simulink model "ABS"  (R2023b)
settings: Solver=FixedStepAuto  StartTime=0.0  StopTime=10  FixedStep=1e-3  MaxStep=1e-3  RelTol=1e-3
values from neighbouring files (symbols this model uses):
  B = 10    [Parameters.m]
  C = 1.9    [Parameters.m]
  D = 1.0    (= 1)    [Parameters.m]
  E = 0.97    [Parameters.m]
  effR = 0.30    (= 0.3)    [Parameters.m]
  g = 9.81    [Parameters.m]
  Jw = 1.8    [Parameters.m]
  lambda_ref = 0.20    (= 0.2)    [Parameters.m]
  omega0 = v0 / effR    (= 92.6)    [Parameters.m]
  QuarterCarMass = 350    [Parameters.m]
  tau_b = 0.03    [Parameters.m]
  Tmax = 2000    [Parameters.m]
  v0 = 27.78    [Parameters.m]
  v_epsilon = 0.5    [Parameters.m]
libraries: slpidlib x1
settings Model: Creator=SEIF  LastModifiedBy=SEIF

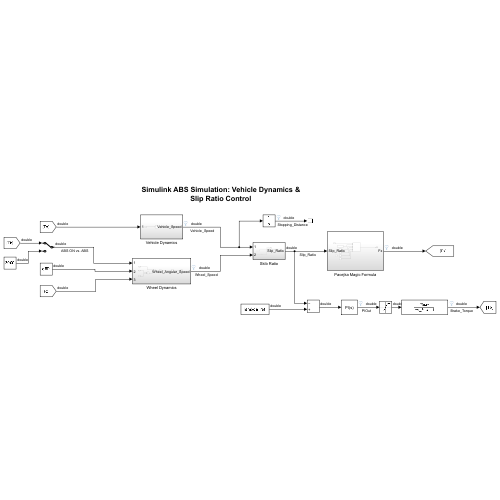
[thumbnail: Simulink's stored preview of the top-level diagram]
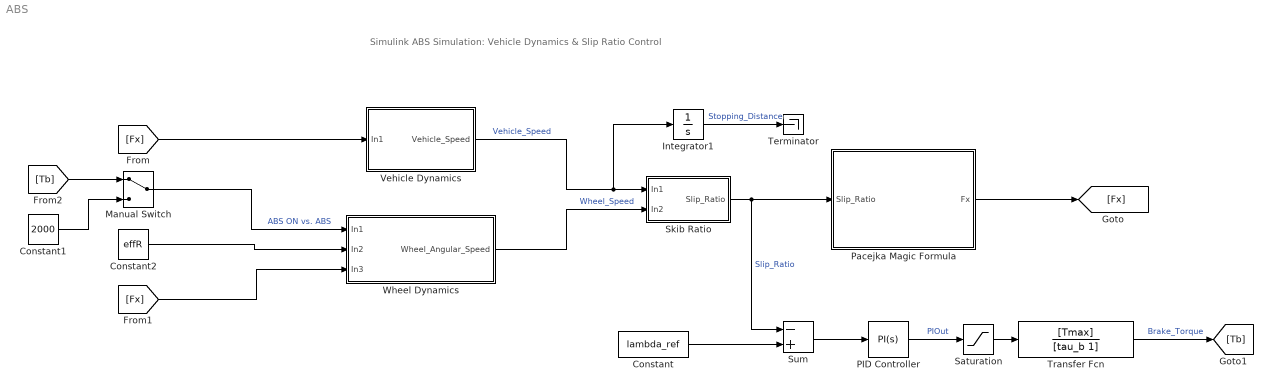
== system ABS ==
  note: Simulink ABS Simulation: Vehicle Dynamics & Slip Ratio Control
  Constant : Constant  Value=lambda_ref
  Constant1 : Constant  Value=2000
  Constant2 : Constant  Value=effR
  Integrator1 : Integrator
  Manual Switch : ManualSwitch
  PID Controller : slpidlib/PID Controller  Controller=PI  Form=Parallel  TimeDomain=Continuous-time  UseExternalTs=off  SampleTime=-1  IntegratorMethod=Forward Euler  FilterMethod=Forward Euler  ControllerParametersSource=internal  P=100  I=10  UseKiTs=off  D=0  N=100  UseFilter=on  TunerSelectOption=Transfer Function Based (PID Tuner App)  InitialConditionSource=internal  InitialConditionForIntegrator=0  InitialConditionForFilter=0  DifferentiatorICPrevScaledInput=0  ExternalReset=none  TrackingMode=off  Kt=1  LimitOutput=off  SatLimitsSource=internal  UpperSaturationLimit=inf  LowerSaturationLimit=-inf  LinearizeAsGain=on  AntiWindupMode=none  Kb=1  LimitIntegrator=off  UpperIntegratorSaturationLimit=inf  LowerIntegratorSaturationLimit=-inf  POutMin=[]  POutMax=[]  IOutMin=[]  IOutMax=[]  DOutMin=[]  DOutMax=[]  NOutMin=[]  NOutMax=[]  SumOutMin=[]  SumOutMax=[]  SaturationOutMin=[]  SaturationOutMax=[]  PParamMin=[]  PParamMax=[]  IParamMin=[]  IParamMax=[]  DParamMin=[]  DParamMax=[]  NParamMin=[]  NParamMax=[]  KbParamMin=[]  KbParamMax=[]  KtParamMin=[]  KtParamMax=[]  KbOutMin=[]  KbOutMax=[]  KtOutMin=[]  KtOutMax=[]  IntegratorOutMin=[]  IntegratorOutMax=[]  FilterOutMin=[]  FilterOutMax=[]  SumI1OutMin=[]  SumI1OutMax=[]  SumI2OutMin=[]  SumI2OutMax=[]  SumI3OutMin=[]  SumI3OutMax=[]  SumI4OutMin=[]  SumI4OutMax=[]  SumDOutMin=[]  SumDOutMax=[]  DifferentiatorOutMin=[]  DifferentiatorOutMax=[]  FilterDiffOutCoefMin=[]  FilterDiffOutCoefMax=[]  ReciprocalOutMin=[]  ReciprocalOutMax=[]  SumDenOutMin=[]  SumDenOutMax=[]  SumNumOutMin=[]  SumNumOutMax=[]  DivideOutMin=[]  DivideOutMax=[]  UdiffTsProdOutMin=[]  UdiffTsProdOutMax=[]  NTsProdOutMin=[]  NTsProdOutMax=[]  UintegralTsProdOutMin=[]  UintegralTsProdOutMax=[]  UngainTsProdOutMin=[]  UngainTsProdOutMax=[]  ClampingZeroOutDataTypeStr=Inherit: Inherit via back propagation  ClampingZeroOutMin=[]  ClampingZeroOutMax=[]  FilterDenConstantOutDataTypeStr=Inherit: Inherit via back propagation  FilterDenConstantOutMin=[]  FilterDenConstantOutMax=[]  PCopyOutDataTypeStr=Inherit: Inherit via back propagation  PCopyOutMin=[]  PCopyOutMax=[]  NCopyOutDataTypeStr=Inherit: Inherit via back propagation  NCopyOutMin=[]  NCopyOutMax=[]  IntegratorContinuousStateAttributes=''  IntegratorStateMustResolveToSignalObject=off  IntegratorRTWStateStorageClass=Auto  FilterContinuousStateAttributes=''  FilterStateMustResolveToSignalObject=off  FilterRTWStateStorageClass=Auto  ParallelPVariant=InternalParameters  IdealPVariant=Disabled  IVariant=InternalParameters  DVariant=Disabled  IntegratorVariant=Continuous  SatVariant=Disabled  AWVariant=Passthrough  PCopyVariant=Disabled  TRVariant=Disabled  FdbkBlocksVariant=Forward  IdealPFdbkVariant=Disabled  SatFdbkVariant=Disabled  DerivativeFilterVariant=Disabled  NVariant=Disabled  NCopyVariant=Disabled_SignalSpec  FilterICVariant=Disabled  IntegratorICVariant=InternalICs  ExternalResetVariant=Disabled  TRSumVariant=Passthrough  SumFdbkVariant=Disabled  SumVariant=Sum_PI  TsampFilterVariant=InternalTs  TsampNgainVariant=Passthrough  TsampIntegralVariant=Disabled_SignalSpec  ExternalSaturationOutDataTypeStr=Inherit: Same as second input
  Pacejka Magic Formula : Subsystem
  Saturation : Saturate  UpperLimit=1  LowerLimit=0
  Skib Ratio : Subsystem
  Sum : Sum  Inputs=-+
  Terminator : Terminator
  Transfer Fcn : TransferFcn  Numerator=[Tmax]  Denominator=[tau_b 1]
  Vehicle Dynamics : Subsystem
  Wheel Dynamics : Subsystem
  wires:
  Pacejka Magic Formula/1(Fx) -> [Fx]
  Constant2/1 -> Wheel Dynamics/2(In2)
  [Fx] -> Wheel Dynamics/3(In3)
  [Fx] -> Vehicle Dynamics/1(In1)
  Wheel Dynamics/1(Wheel_Angular_Speed) -> Skib Ratio/2(In2)  "Wheel_Speed"
  Skib Ratio/1(Slip_Ratio) -> Sum/1, Pacejka Magic Formula/1(Slip_Ratio)  "Slip_Ratio"
  Constant/1 -> Sum/2
  Sum/1 -> PID Controller/1
  PID Controller/1 -> Saturation/1  "PIOut"
  Saturation/1 -> Transfer Fcn/1
  Transfer Fcn/1 -> [Tb]  "Brake_Torque"
  Integrator1/1 -> Terminator/1  "Stopping_Distance"
  Vehicle Dynamics/1(Vehicle_Speed) -> Integrator1/1, Skib Ratio/1(In1)  "Vehicle_Speed"
  Manual Switch/1 -> Wheel Dynamics/1(In1)  "ABS ON vs. ABS"
  [Tb] -> Manual Switch/1
  Constant1/1 -> Manual Switch/2

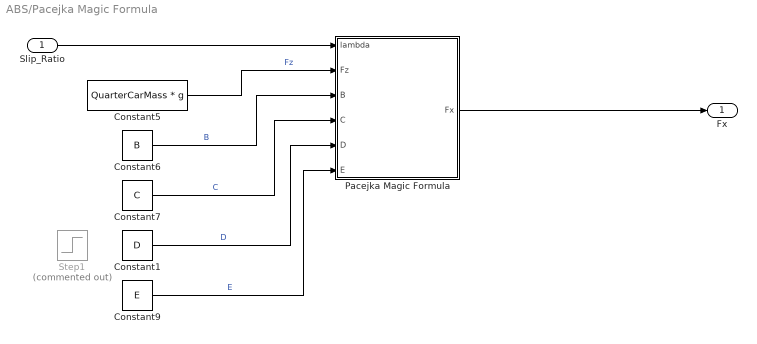
== system ABS/Pacejka Magic Formula ==
  Slip_Ratio : Inport
  Constant1 : Constant  Value=D
  Constant5 : Constant  Value=QuarterCarMass * g
  Constant6 : Constant  Value=B
  Constant7 : Constant  Value=C
  Constant9 : Constant  Value=E
  Pacejka Magic Formula : MATLAB Function  TreatAsAtomicUnit=on
  Step1 : Step  Commented=on  Before=1  After=0.4  SampleTime=0
  Fx : Outport
  wires:
  Slip_Ratio/1 -> Pacejka Magic Formula/1(lambda)
  Constant7/1 -> Pacejka Magic Formula/4(C)  "C"
  Constant5/1 -> Pacejka Magic Formula/2(Fz)  "Fz"
  Constant9/1 -> Pacejka Magic Formula/6(E)  "E"
  Constant6/1 -> Pacejka Magic Formula/3(B)  "B"
  Constant1/1 -> Pacejka Magic Formula/5(D)  "D"
  Pacejka Magic Formula/1(Fx) -> Fx/1

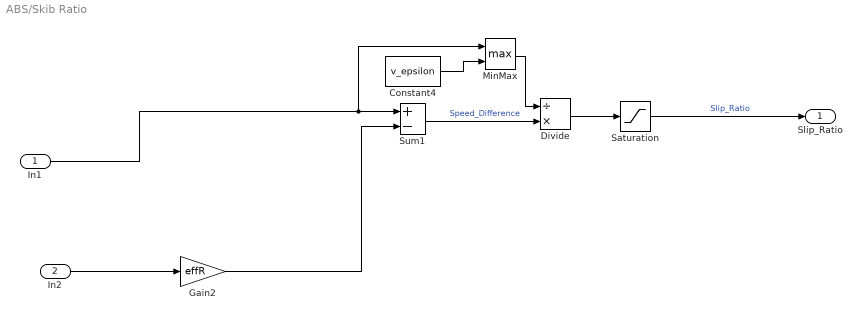
== system ABS/Skib Ratio ==
  In1 : Inport
  In2 : Inport  Port=2
  Constant4 : Constant  Value=v_epsilon
  Divide : Product  Inputs=/*
  Gain2 : Gain  Gain=effR
  MinMax : MinMax  Function=max  Inputs=2
  Saturation : Saturate  UpperLimit=1  LowerLimit=0
  Sum1 : Sum  Inputs=+-
  Slip_Ratio : Outport
  wires:
  Gain2/1 -> Sum1/2
  Saturation/1 -> Slip_Ratio/1  "Slip_Ratio"
  Sum1/1 -> Divide/2  "Speed_Difference"
  In1/1 -> MinMax/1, Sum1/1
  Constant4/1 -> MinMax/2
  MinMax/1 -> Divide/1
  Divide/1 -> Saturation/1
  In2/1 -> Gain2/1

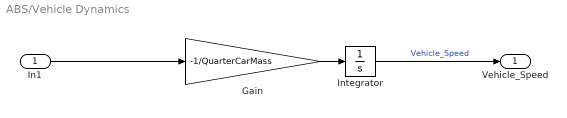
== system ABS/Vehicle Dynamics ==
  In1 : Inport
  Gain : Gain  Gain=-1/QuarterCarMass
  Integrator : Integrator  InitialCondition=v0  LimitOutput=on  LowerSaturationLimit=0
  Vehicle_Speed : Outport
  wires:
  Gain/1 -> Integrator/1
  Integrator/1 -> Vehicle_Speed/1  "Vehicle_Speed"
  In1/1 -> Gain/1

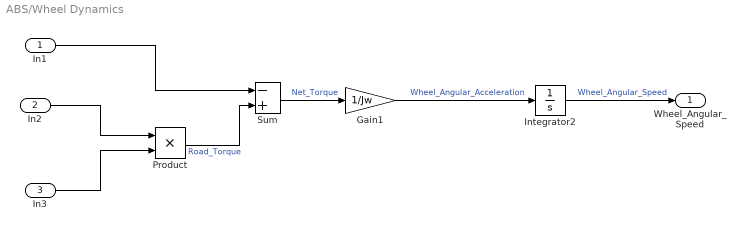
== system ABS/Wheel Dynamics ==
  In1 : Inport
  In2 : Inport  Port=2
  In3 : Inport  Port=3
  Gain1 : Gain  Gain=1/Jw
  Integrator2 : Integrator  InitialCondition=omega0  LimitOutput=on  LowerSaturationLimit=0
  Product : Product
  Sum : Sum  Inputs=-+
  Wheel_Angular_Speed : Outport
  wires:
  In1/1 -> Sum/1
  Sum/1 -> Gain1/1  "Net_Torque"
  Gain1/1 -> Integrator2/1  "Wheel_Angular_Acceleration"
  Product/1 -> Sum/2  "Road_Torque"
  Integrator2/1 -> Wheel_Angular_Speed/1  "Wheel_Angular_Speed"
  In2/1 -> Product/1
  In3/1 -> Product/2

== matlab function ABS/Pacejka Magic Formula/Pacejka Magic Formula ==
  data: lambda input; Fx output; Fz input; B input; C input; D input; E input
function Fx = fcn(lambda, Fz, B, C, D, E)

    mu = D * sin(C * atan(B * lambda - E * (B * lambda - atan(B * lambda))));
    Fx = mu * Fz;
    
end
